simulink model "OFDMmodel_synch_18B1"  (R2025b)
settings: Solver=VariableStepAuto  StartTime=0.0  StopTime=inf  RelTol=1e-3
values from neighbouring files (symbols this model uses):
  BandasG = NFFT/4-4    (= 12)    [InitOFDM.m]
  Carriers = 1:NFFT    [InitOFDM.m]
  ChannEstData = PHI(DataCarrierIn,:)*Ainv    [InitOFDM.m]
  CP = 16    [InitOFDM.m]    (also in OFDMwideband_BEM2D.m = 32)
  DataCarrierIn = Carriers    [InitOFDM.m]
  DataCarriers = numel(DataCarrierIn)    [InitOFDM.m]
  DataCarriersFrame = DataCarriers*FrameSize    [InitOFDM.m]
  FrameSize = 40    [InitOFDM.m]
  FrameTime = Tsymbol*(FrameSize+2)    (= 0.000168)    [InitOFDM.m]
  NFFT = 64    [InitOFDM.m]    (also in OFDMwideband_BEM2D.m = 256)
  PilotIndex = UsedIndex(2:floor(numel(UsedIndex)/10):end)    [InitOFDM.m]
  pilots = randsrc(numel(PilotIndex),1,[-1 1 1i 1i])*.71    [InitOFDM.m]
  PreambuloFrec = zeros(64,1)    [InitOFDM.m]    (also in Preambulo.mat = [0 0 0 0 0 0 0 0 4 0 0 0 ... (64 elements, 64x1)])
  Ts = 1/Fs    (= 5e-08)    [InitOFDM.m]    (also in OFDMwideband_BEM2D.m = 1e-07)
undefined symbols (not defined in the file or in its folder): get, ifftshift, jet, LogicIndex, Low, magnitude
libraries: simulink x5, dspsigops x5, dspxfrm3 x4, commrflib2 x2, commchan3 x1, dspobslib x1, commrandsrc3 x1, commdigbbndam3 x1, dspswit3 x1, dspmathops x1
settings Model: Creator=Fernando  LastModifiedBy=gonzalogutierrez
settings SolverCC: AlgebraicLoopSolver=TrustRegion
settings DataIOCC: LimitDataPoints=on  MaxDataPoints=1  DSMLogging=off  SaveTime=off
settings DebuggingCC: UnconnectedInputMsg=warning  UnconnectedOutputMsg=warning  UnconnectedLineMsg=warning  ArithmeticOperatorsInVariantConditions=warning
settings ModelReferenceCC: EnableRefExpFcnMdlSchedulingChecks=on
settings SFSimCC: CustomCodeUndefinedFunction=UseInterfaceOnly
settings RTWCC: GPUComputeCapability=3.5

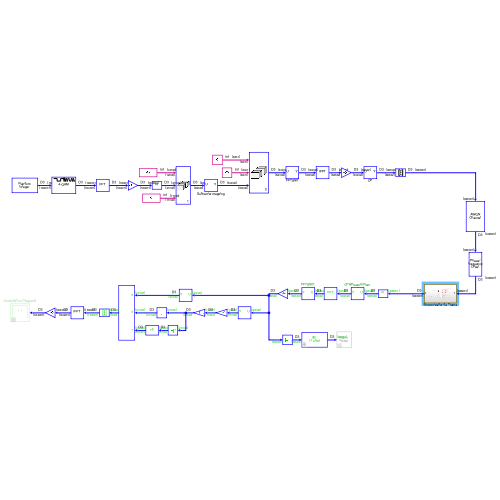
[thumbnail: Simulink's stored preview of the top-level diagram]
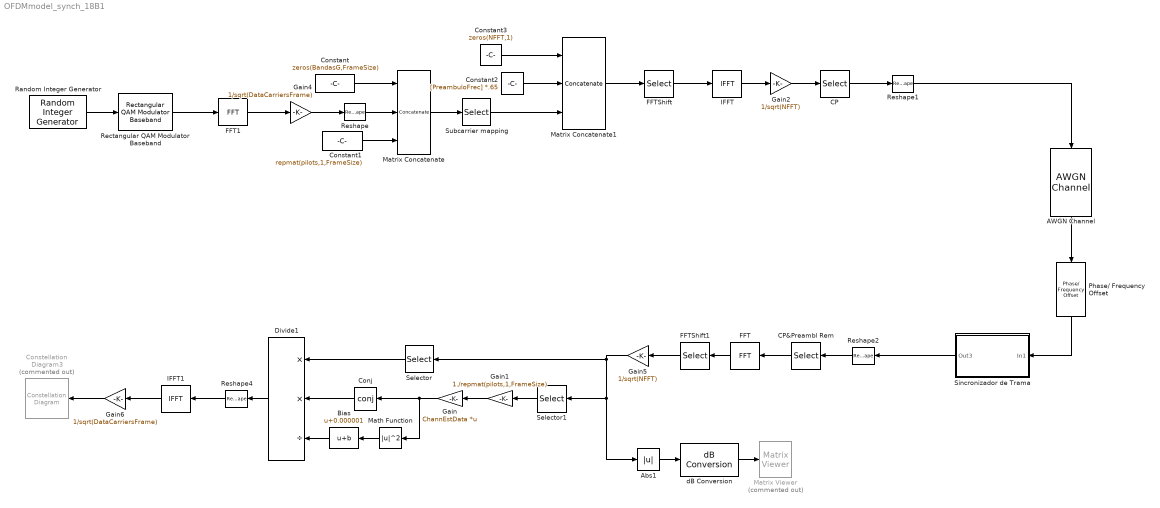
== system OFDMmodel_synch_18B1 ==
  AWGN Channel : commchan3/AWGN Channel  LegacyMode=on  NoiseMethod="Signal to noise ratio  (SNR)"  noiseMode="Signal to noise ratio  (SNR)"  EbNo=10  EsNo=10  SNR=30  BitsPerSymbol=1  SignalPower=1  SpecifySymbolPeriod=off  SamplesPerSymbol=1  SymbolPeriod=1  VarianceSource=Parameter  Variance=1  RandomStream=Global stream  Seed=67  SimulateUsing=Code generation
  Abs1 : Abs  SaturateOnIntegerOverflow=off
  Bias : Bias  Bias=0.000001  SaturateOnIntegerOverflow=off
  CP : Selector  NumberOfDimensions=2  InputPortWidth=NFFT  IndexOptions=Index vector (dialog),Select all  Indices=[NFFT-CP+1:NFFT 1:NFFT],1  OutputSizes=1,1
  CP&Preambl Rem : Selector  NumberOfDimensions=2  InputPortWidth=NFFT+CP  IndexOptions=Starting index (dialog),Starting index (dialog)  Indices=CP+1,2  OutputSizes=NFFT,FrameSize
  Conj : Math  Operator=conj  SignedPower=on
  Constant : Constant  Value=zeros(BandasG,FrameSize)  VectorParams1D=off
  Constant1 : Constant  Value=repmat(pilots,1,FrameSize)  VectorParams1D=off
  Constant2 : Constant  Value=[PreambuloFrec] *.65  VectorParams1D=off
  Constant3 : Constant  Value=zeros(NFFT,1)  VectorParams1D=off
  Constellation Diagram3 : ConstellationDiagram  Commented=on  DefaultConfigurationName=comm.scopes.ConstellationDiagramBlockCfg
  Divide1 : Product  Inputs=**/
  FFT : dspxfrm3/FFT  FFTImplementation=Auto  CompMethod=Table lookup  TableOpt=NEW  TableOptActive=Speed  BitRevOrder=off  Normalize=off  InheritFFTLength=on  FFTLength=64  WrapInput=on  roundingMode=Floor  overflowMode=off  firstCoeffDataTypeStr=Inherit: Same word length as input  firstCoeffLastDataTypeStr=Inherit: Same word length as input  outputMin=[]  outputMax=[]
  FFT1 : dspxfrm3/FFT  FFTImplementation=Auto  CompMethod=Table lookup  TableOpt=NEW  TableOptActive=Speed  BitRevOrder=off  Normalize=off  InheritFFTLength=on  FFTLength=64  WrapInput=on  roundingMode=Floor  overflowMode=off  firstCoeffDataTypeStr=Inherit: Same word length as input  firstCoeffLastDataTypeStr=Inherit: Same word length as input  outputMin=[]  outputMax=[]
  FFTShift : Selector  NumberOfDimensions=2  InputPortWidth=NFFT  IndexOptions=Index vector (dialog),Select all  Indices=ifftshift(Carriers),1  OutputSizes=1,1
  FFTShift1 : Selector  NumberOfDimensions=2  InputPortWidth=NFFT  IndexOptions=Index vector (dialog),Select all  Indices=ifftshift(Carriers),1  OutputSizes=1,1
  Gain : Gain  Gain=ChannEstData  Multiplication=Matrix(K*u)
  Gain1 : Gain  Gain=1./repmat(pilots,1,FrameSize)
  Gain2 : Gain  Gain=1/sqrt(NFFT)
  Gain4 : Gain  Gain=1/sqrt(DataCarriersFrame)
  Gain5 : Gain  Gain=1/sqrt(NFFT)
  Gain6 : Gain  Gain=1/sqrt(DataCarriersFrame)
  IFFT : dspxfrm3/IFFT  FFTImplementation=Auto  CompMethod=Table lookup  TableOpt=NEW  TableOptActive=Speed  BitRevOrder=off  cs_in=off  Normalize=off  InheritFFTLength=on  FFTLength=64  WrapInput=on  mode=Complex  outSamplingMode=Sample based  roundingMode=Floor  overflowMode=off  firstCoeffDataTypeStr=Inherit: Same word length as input  firstCoeffLastDataTypeStr=Inherit: Same word length as input  outputMin=[]  outputMax=[]
  IFFT1 : dspxfrm3/IFFT  FFTImplementation=Auto  CompMethod=Table lookup  TableOpt=NEW  TableOptActive=Speed  BitRevOrder=off  cs_in=off  Normalize=off  InheritFFTLength=on  FFTLength=64  WrapInput=on  mode=Complex  outSamplingMode=Sample based  roundingMode=Floor  overflowMode=off  firstCoeffDataTypeStr=Inherit: Same word length as input  firstCoeffLastDataTypeStr=Inherit: Same word length as input  outputMin=[]  outputMax=[]
  Math Function : Math  Operator=magnitude^2  SignedPower=on
  Matrix Concatenate : Concatenate  NumInputs=3  Mode=Multidimensional array
  Matrix Concatenate1 : Concatenate  NumInputs=3  Mode=Multidimensional array  ConcatenateDimension=2
  Matrix Viewer : dspobslib/Matrix Viewer  Commented=on  ImageParams=off  CMapStr=jet(256)  AxisColorbar=on  AxisParams=off  AxisOrigin=Upper left corner  AxisTickMode=Auto  XTickRange=[0 1]  YTickRange=[0 1]  XLabel=X-axis  YLabel=Y-axis  ZLabel=Z-axis  FigPos=get(0,'defaultfigureposition')  AxisZoom=off
      settings: YMin=-30  YMax=-20
  Phase/ Frequency Offset : commrflib2/Phase// Frequency Offset  phaseOffset=0  freqPort=off  freqOffset=5e3
  Random Integer Generator : commrandsrc3/Random Integer Generator  SetSize=ConstSize  SeedSource=Auto  Seed=0  SampleTime=FrameTime/(DataCarriers*FrameSize)  SamplesPerFrame=DataCarriers*FrameSize  OutputDataType=double  SimulateUsing=Interpreted execution
  Rectangular QAM Modulator Baseband : commdigbbndam3/Rectangular QAM Modulator Baseband  M=ConstSize  InType=Integer  Enc=Gray  Mapping=[0:15]  PowType=Average Power  MinDist=2  AvgPow=1  PeakPow=1  Ph=0  outDtype=double  outWordLen=16  outUDDataType=sfix(16)  outFracLenMode=Best precision  outFracLen=15  outDataTypeStr=double  outLastDataTypeStr=double
  Reshape : Reshape  OutputDimensionality=Customize  OutputDimensions=[DataCarriers,FrameSize]
  Reshape1 : Reshape  OutputDimensionality=Column vector (2-D)  OutputDimensions=[DataCarriers,FrameSize]
  Reshape2 : Reshape  OutputDimensionality=Customize  OutputDimensions=[NFFT+CP,FrameSize+2]
  Reshape4 : Reshape  OutputDimensionality=Column vector (2-D)  OutputDimensions=[DataCarriers,FrameSize]
  Selector : Selector  NumberOfDimensions=2  InputPortWidth=NFFT  IndexOptions=Index vector (dialog),Select all  Indices=DataCarrierIn,1  OutputSizes=1,1
  Selector1 : Selector  NumberOfDimensions=2  InputPortWidth=NFFT  IndexOptions=Index vector (dialog),Select all  Indices=PilotIndex,1  OutputSizes=1,1
  Sincronizador de Trama : Subsystem
  Subcarrier mapping : Selector  NumberOfDimensions=2  InputPortWidth=NFFT  IndexOptions=Index vector (dialog),Select all  Indices=LogicIndex,1  OutputSizes=1,1
  dB Conversion : dspmathops/dB Conversion  dBtype=dB  intype=Amplitude  R=1  fuzz=off
  wires:
  Constant/1 -> Matrix Concatenate/1
  Matrix Concatenate/1 -> Subcarrier mapping/1
  IFFT/1 -> Gain2/1
  CP/1 -> Reshape1/1
  Constant1/1 -> Matrix Concatenate/3
  Selector1/1 -> Gain1/1
  Selector/1 -> Divide1/1
  Random Integer Generator/1 -> Rectangular QAM Modulator Baseband/1
  Gain2/1 -> CP/1
  FFT/1 -> FFTShift1/1
  FFTShift1/1 -> Gain5/1
  Conj/1 -> Divide1/2
  Gain/1 -> Math Function/1, Conj/1
  Bias/1 -> Divide1/3
  Math Function/1 -> Bias/1
  Divide1/1 -> Reshape4/1
  CP&Preambl Rem/1 -> FFT/1
  Reshape/1 -> Matrix Concatenate/2
  Abs1/1 -> dB Conversion/1
  Matrix Concatenate1/1 -> FFTShift/1
  FFTShift/1 -> IFFT/1
  Constant2/1 -> Matrix Concatenate1/2
  Constant3/1 -> Matrix Concatenate1/1
  dB Conversion/1 -> Matrix Viewer/1
  Gain5/1 -> Selector1/1, Abs1/1, Selector/1
  Gain1/1 -> Gain/1
  Rectangular QAM Modulator Baseband/1 -> FFT1/1
  FFT1/1 -> Gain4/1
  IFFT1/1 -> Gain6/1
  Gain4/1 -> Reshape/1
  Gain6/1 -> Constellation Diagram3/1
  Reshape4/1 -> IFFT1/1
  Reshape2/1 -> CP&Preambl Rem/1
  Subcarrier mapping/1 -> Matrix Concatenate1/3
  Reshape1/1 -> AWGN Channel/1
  AWGN Channel/1 -> Phase/ Frequency Offset/1
  Phase/ Frequency Offset/1 -> Sincronizador de Trama/1(In1)
  Sincronizador de Trama/1(Out3) -> Reshape2/1

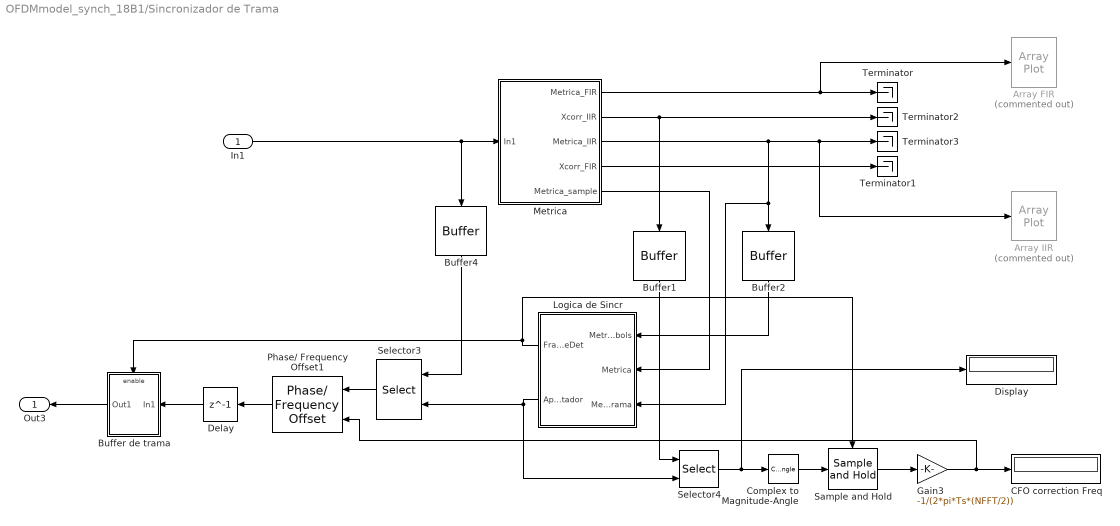
== system OFDMmodel_synch_18B1/Sincronizador de Trama ==
  In1 : Inport
  Array FIR : ArrayPlot  Commented=on  WindowPosition=[481 42 958 954]  AxesScaling=Manual  YLimits=[-0.125,1.125]  ShowGrid=off  ChannelNames="[\"\"]"  DefaultConfigurationName=dsp.scopes.ArrayPlotBlockSpecification
  Array IIR : ArrayPlot  Commented=on  WindowPosition=[241.000000,-27.000000,958.000000,954.000000,]  ScopeFrameLocation=window  AxesScaling=Manual  YLimits=[-0.125,1.125]  ShowGrid=off  ChannelNames="[\"\"]"  DefaultConfigurationName=dsp.scopes.ArrayPlotBlockSpecification
  Buffer de trama : Subsystem
  Buffer1 : Buffer  N=2*(NFFT+CP)  V=NFFT+CP  OutputFrames=off
  Buffer2 : Buffer  N=2*(NFFT+CP)  V=NFFT+CP  OutputFrames=off
  Buffer4 : Buffer  N=3*(NFFT+CP)  V=2*(NFFT+CP)  OutputFrames=off
  CFO correction Freq : Display
  Complex to Magnitude-Angle : ComplexToMagnitudeAngle  Output=Angle
  Delay : Delay  DelayLength=1
  Display : Display
  Gain3 : Gain  Gain=-1/(2*pi*Ts*(NFFT/2))
  Logica de Sincr : Subsystem
  Metrica : Subsystem
  Phase/ Frequency Offset1 : commrflib2/Phase// Frequency Offset  phaseOffset=0  freqPort=on  freqOffset=16e3
  Sample and Hold : dspsigops/Sample and Hold  trig=Rising edge  initCond=0  latchinput=off
  Selector3 : Selector  InputPortWidth=3*(NFFT+CP)  IndexOptions=Starting index (port)  Indices=[1 3]  OutputSizes=NFFT+CP
  Selector4 : Selector  InputPortWidth=2*(NFFT+CP)  IndexOptions=Index vector (port)  Indices=[1 3]  OutputSizes=1
  Terminator{,1..3} (4 alike) : Terminator
  Out3 : Outport
  wires:
  Phase/ Frequency Offset1/1 -> Delay/1
  Gain3/1 -> Phase/ Frequency Offset1/2, CFO correction Freq/1
  Buffer1/1 -> Selector4/1
  Logica de Sincr/2(Apuntador) -> Selector4/2, Selector3/2
  Sample and Hold/1 -> Gain3/1
  Logica de Sincr/1(FrameDet) -> Buffer de trama/Enable, Sample and Hold/Trigger
  Buffer4/1 -> Selector3/1
  Buffer2/1 -> Logica de Sincr/1(Metrica_2Symbols)
  Complex to Magnitude-Angle/1 -> Sample and Hold/1
  Selector3/1 -> Phase/ Frequency Offset1/1
  Metrica/2(Xcorr_IIR) -> Buffer1/1, Terminator2/1
  Delay/1 -> Buffer de trama/1(In1)
  Selector4/1 -> Display/1, Complex to Magnitude-Angle/1
  In1/1 -> Metrica/1(In1), Buffer4/1
  Metrica/3(Metrica_IIR) -> Logica de Sincr/3(Metrica_trama), Buffer2/1, Array IIR/1, Terminator3/1
  Buffer de trama/1(Out1) -> Out3/1
  Metrica/4(Xcorr_FIR) -> Terminator1/1
  Metrica/1(Metrica_FIR) -> Terminator/1, Array FIR/1
  Metrica/5(Metrica_sample) -> Logica de Sincr/2(Metrica)

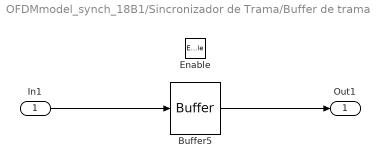
== system OFDMmodel_synch_18B1/Sincronizador de Trama/Buffer de trama ==
  In1 : Inport
  Enable : EnablePort  ZeroCross=off
  Buffer5 : Buffer  N=(NFFT+CP)*(FrameSize+2)  OutputFrames=off
  Out1 : Outport
  wires:
  In1/1 -> Buffer5/1
  Buffer5/1 -> Out1/1

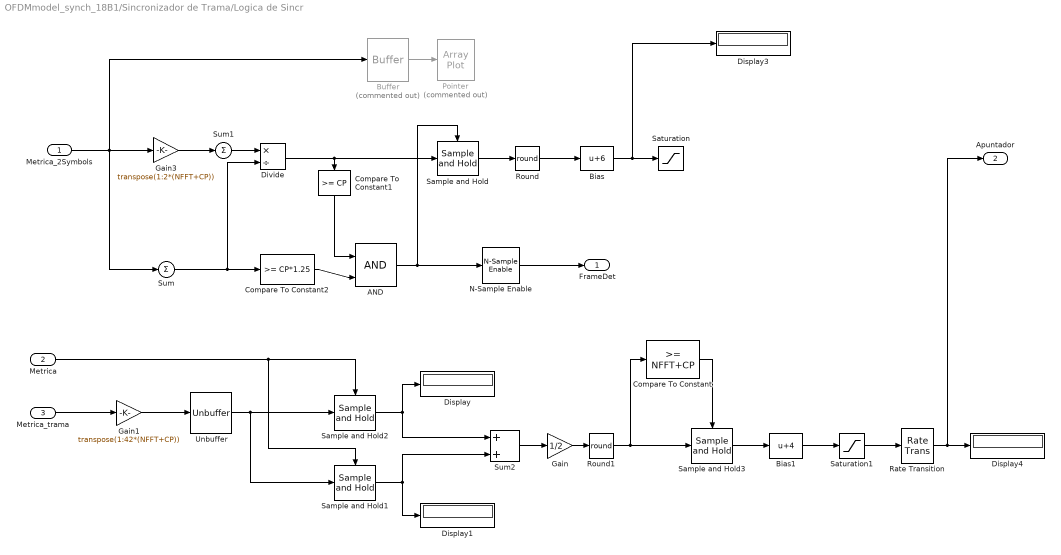
== system OFDMmodel_synch_18B1/Sincronizador de Trama/Logica de Sincr ==
  Metrica_2Symbols : Inport
  Metrica : Inport  Port=2
  Metrica_trama : Inport  Port=3
  AND : Logic  IconShape=distinctive  AllPortsSameDT=off  OutDataTypeStr=boolean
  Bias : Bias  Bias=6  SaturateOnIntegerOverflow=off
  Bias1 : Bias  Bias=4  SaturateOnIntegerOverflow=off
  Buffer : Buffer  Commented=on  N=2*(NFFT + CP)  OutputFrames=off
  Compare To Constant : simulink/Logic and Bit Operations/Compare To Constant  relop=>=  const=NFFT+CP  OutDataTypeStr=boolean
  Compare To Constant1 : simulink/Logic and Bit Operations/Compare To Constant  relop=>=  const=CP  OutDataTypeStr=boolean  ZeroCross=off
  Compare To Constant2 : simulink/Logic and Bit Operations/Compare To Constant  relop=>=  const=CP*1.25  OutDataTypeStr=boolean  ZeroCross=off
  Display{,1,3..4} (4 alike) : Display
  Divide : Product  Inputs=*/
  Gain : Gain  Gain=1/2
  Gain1 : Gain  Gain=transpose(1:42*(NFFT+CP))
  Gain3 : Gain  Gain=transpose(1:2*(NFFT+CP))
  N-Sample Enable : dspswit3/N-Sample Enable  N=FrameSize+1  ActiveLevel=Low (0)  reset=on  TriggerType=Rising edge  Ts=1  DataType=Logical
  Pointer : ArrayPlot  Commented=on  WindowPosition=[481 42 958 954]  AxesScaling=Manual  YLimits=[-16.5,168.5]  ShowGrid=off  ChannelNames="[\"\"]"  DefaultConfigurationName=dsp.scopes.ArrayPlotBlockSpecification
  Rate Transition : RateTransition  OutPortSampleTime=4e-6
  Round : Rounding  Operator=round
  Round1 : Rounding  Operator=round
  Sample and Hold : dspsigops/Sample and Hold  trig=Rising edge  initCond=0  latchinput=off
  Sample and Hold1 : dspsigops/Sample and Hold  trig=Falling edge  initCond=0  latchinput=off
  Sample and Hold2 : dspsigops/Sample and Hold  trig=Rising edge  initCond=0  latchinput=off
  Sample and Hold3 : dspsigops/Sample and Hold  trig=Rising edge  initCond=0  latchinput=off
  Saturation : Saturate  UpperLimit=2*(NFFT+CP)+1  LowerLimit=1
  Saturation1 : Saturate  UpperLimit=2*(NFFT+CP)+1  LowerLimit=1
  Sum : Sum  Inputs=+
  Sum1 : Sum  Inputs=+
  Sum2 : Sum
  Unbuffer : Unbuffer
  FrameDet : Outport
  Apuntador : Outport  Port=2
  wires:
  Metrica_2Symbols/1 -> Sum/1, Buffer/1, Gain3/1
  Sum/1 -> Divide/2, Compare To Constant2/1
  Gain3/1 -> Sum1/1
  AND/1 -> Sample and Hold/Trigger, N-Sample Enable/1
  Round/1 -> Bias/1
  Sample and Hold/1 -> Round/1
  Sum1/1 -> Divide/1
  N-Sample Enable/1 -> FrameDet/1
  Bias/1 -> Display3/1, Saturation/1
  Compare To Constant2/1 -> AND/2
  Compare To Constant1/1 -> AND/1
  Buffer/1 -> Pointer/1
  Divide/1 -> Sample and Hold/1, Compare To Constant1/1
  Metrica_trama/1 -> Gain1/1
  Sample and Hold1/1 -> Sum2/2, Display1/1
  Sample and Hold2/1 -> Sum2/1, Display/1
  Metrica/1 -> Sample and Hold2/Trigger, Sample and Hold1/Trigger
  Sum2/1 -> Gain/1
  Gain1/1 -> Unbuffer/1
  Unbuffer/1 -> Sample and Hold1/1, Sample and Hold2/1
  Gain/1 -> Round1/1
  Sample and Hold3/1 -> Bias1/1
  Compare To Constant/1 -> Sample and Hold3/Trigger
  Round1/1 -> Compare To Constant/1, Sample and Hold3/1
  Bias1/1 -> Saturation1/1
  Saturation1/1 -> Rate Transition/1
  Rate Transition/1 -> Apuntador/1, Display4/1

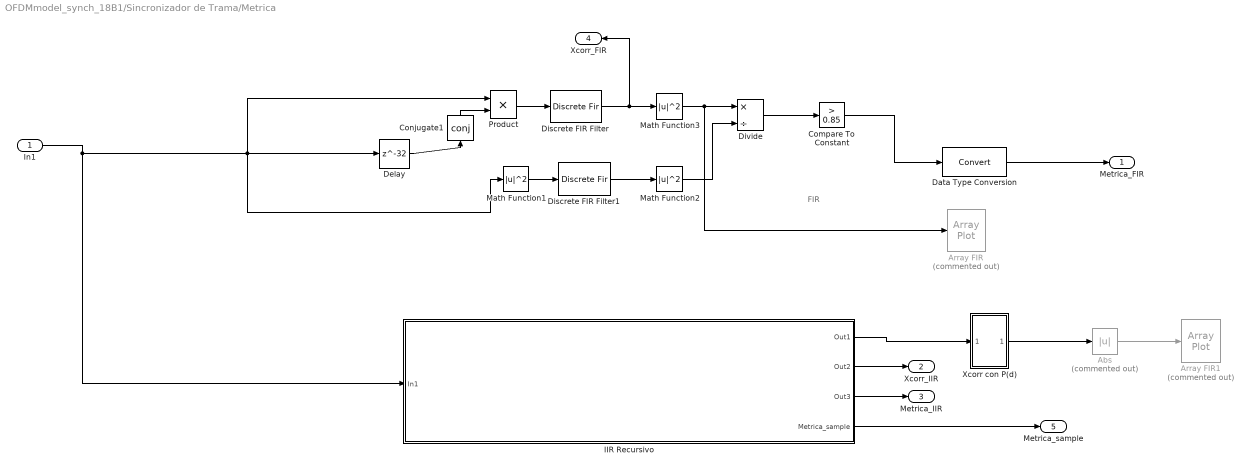
== system OFDMmodel_synch_18B1/Sincronizador de Trama/Metrica ==
  note: FIR
  In1 : Inport
  Abs : Abs  Commented=on  SaturateOnIntegerOverflow=off
  Array FIR : ArrayPlot  Commented=on  WindowPosition=[480 -51 958 954]  AxesScaling=Manual  YLimits=[-821.624,7394.62]  ShowGrid=off  ChannelNames="[\"\"]"  DefaultConfigurationName=dsp.scopes.ArrayPlotBlockSpecification
  Array FIR1 : ArrayPlot  Commented=on  WindowPosition=[2 -5 1920 963]  AxesScaling=Manual  YLimits=[-16377.7,109222]  ShowGrid=off  ChannelNames="[\"\"]"  DefaultConfigurationName=dsp.scopes.ArrayPlotBlockSpecification
  Compare To Constant : simulink/Logic and Bit Operations/Compare To Constant  relop=>  const=0.85  OutDataTypeStr=uint8  ZeroCross=off
  Conjugate1 : Math  Operator=conj  SignedPower=on  RndMeth=Zero
  Data Type Conversion : DataTypeConversion  SaturateOnIntegerOverflow=off  RndMeth=Floor
  Delay : Delay  DelayLength=32  InputProcessing=Columns as channels (frame based)
  Discrete FIR Filter : DiscreteFir  Coefficients=ones(1,32)  InputProcessing=Columns as channels (frame based)
  Discrete FIR Filter1 : DiscreteFir  Coefficients=0.5*ones(1,NFFT)  InputProcessing=Columns as channels (frame based)
  Divide : Product  Inputs=*/
  IIR Recursivo : Subsystem
  Math Function1 : Math  Operator=magnitude^2  SignedPower=on
  Math Function2 : Math  Operator=magnitude^2  SignedPower=on
  Math Function3 : Math  Operator=magnitude^2  SignedPower=on
  Product : Product
  Xcorr con P(d) : Subsystem
  Metrica_FIR : Outport
  Xcorr_IIR : Outport  Port=2
  Metrica_IIR : Outport  Port=3
  Xcorr_FIR : Outport  Port=4
  Metrica_sample : Outport  Port=5
  wires:
  Delay/1 -> Conjugate1/1
  Discrete FIR Filter/1 -> Xcorr_FIR/1, Math Function3/1
  Product/1 -> Discrete FIR Filter/1
  Math Function1/1 -> Discrete FIR Filter1/1
  Compare To Constant/1 -> Data Type Conversion/1
  Discrete FIR Filter1/1 -> Math Function2/1
  Math Function3/1 -> Array FIR/1, Divide/1
  Math Function2/1 -> Divide/2
  Data Type Conversion/1 -> Metrica_FIR/1
  Conjugate1/1 -> Product/2
  Divide/1 -> Compare To Constant/1
  In1/1 -> IIR Recursivo/1(In1), Product/1, Delay/1, Math Function1/1
  IIR Recursivo/1(Out1) -> Xcorr con P(d)/1(In1)
  IIR Recursivo/2(Out2) -> Xcorr_IIR/1
  IIR Recursivo/3(Out3) -> Metrica_IIR/1
  Xcorr con P(d)/1(Out1) -> Abs/1
  Abs/1 -> Array FIR1/1
  IIR Recursivo/4(Metrica_sample) -> Metrica_sample/1

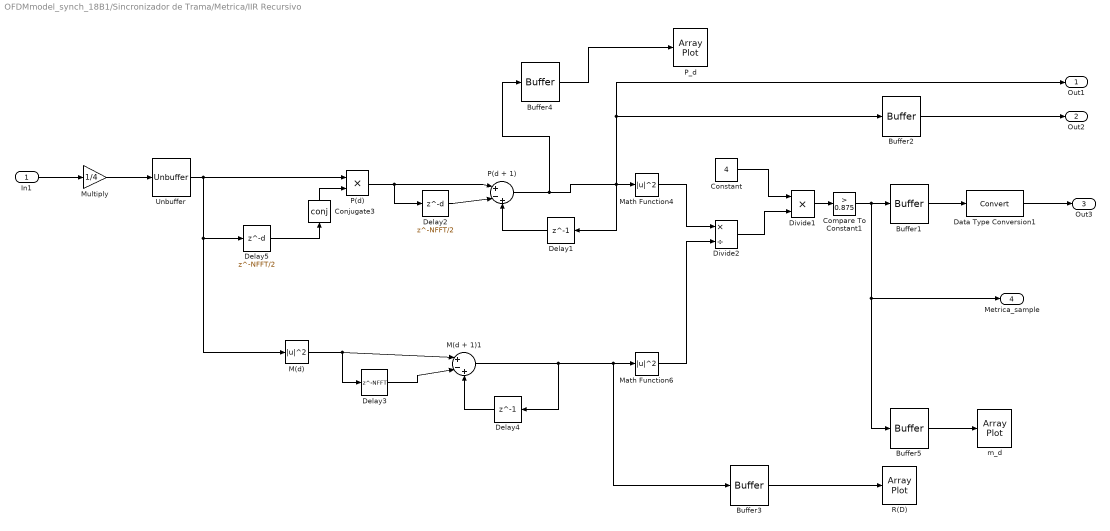
== system OFDMmodel_synch_18B1/Sincronizador de Trama/Metrica/IIR Recursivo ==
  In1 : Inport
  Buffer{1..5} (5 alike) : Buffer  N=(NFFT + CP) * 42  OutputFrames=off
  Compare To Constant1 : simulink/Logic and Bit Operations/Compare To Constant  relop=>  const=0.875  OutDataTypeStr=uint8  ZeroCross=off
  Conjugate3 : Math  Operator=conj  SignedPower=on  RndMeth=Zero
  Constant : Constant  Value=4
  Data Type Conversion1 : DataTypeConversion  SaturateOnIntegerOverflow=off  RndMeth=Floor
  Delay1 : Delay  DelayLength=1
  Delay2 : Delay  DelayLength=NFFT/2  InputProcessing=Columns as channels (frame based)
  Delay3 : Delay  DelayLength=NFFT
  Delay4 : Delay  DelayLength=1
  Delay5 : Delay  DelayLength=NFFT/2  InputProcessing=Columns as channels (frame based)
  Divide1 : Product  Inputs=**
  Divide2 : Product  Inputs=*/
  M(d + 1)1 : Sum  Inputs=|+-+
  M(d) : Math  Operator=magnitude^2  SignedPower=on
  Math Function4 : Math  Operator=magnitude^2  SignedPower=on
  Math Function6 : Math  Operator=magnitude^2  SignedPower=on
  Multiply : Gain  Gain=1/4
  P(d + 1) : Sum  Inputs=|+-+
  P(d) : Product
  P_d : ArrayPlot  WindowPosition=[0.000000,1.000000,1440.000000,842.000000,]  Visible=on  ScopeFrameLocation=window  AxesScaling=Manual  MaximizeAxes=Off  YLimits=[-0.9249 5.7278]  ShowGrid=off  ChannelNames="[\"\"]"  DefaultConfigurationName=dsp.scopes.ArrayPlotBlockSpecification
  R(D) : ArrayPlot  WindowPosition=[721.000000,1.000000,720.000000,842.000000,]  Visible=on  ScopeFrameLocation=window  AxesScaling=Manual  YLimits=[7.313850160256411 10.478150160256412]  ShowGrid=off  ChannelNames="[\"\"]"  DefaultConfigurationName=dsp.scopes.ArrayPlotBlockSpecification
  Unbuffer : Unbuffer
  m_d : ArrayPlot  WindowPosition=[1.000000,1.000000,1440.000000,842.000000,]  Visible=on  ScopeFrameLocation=window  AxesScaling=Manual  YLimits=[-0.116212,1.04604]  ShowGrid=off  ChannelNames="[\"\"]"  DefaultConfigurationName=dsp.scopes.ArrayPlotBlockSpecification
  Out1 : Outport
  Out2 : Outport  Port=2
  Out3 : Outport  Port=3
  Metrica_sample : Outport  Port=4
  wires:
  P(d + 1)/1 -> Buffer4/1, Out1/1, Buffer2/1, Math Function4/1, Delay1/1
  M(d)/1 -> Delay3/1, M(d + 1)1/1
  Unbuffer/1 -> P(d)/1, M(d)/1, Delay5/1
  Delay4/1 -> M(d + 1)1/3
  Buffer1/1 -> Data Type Conversion1/1
  Math Function6/1 -> Divide2/2
  P(d)/1 -> Delay2/1, P(d + 1)/1
  Compare To Constant1/1 -> Buffer5/1, Metrica_sample/1, Buffer1/1
  Divide2/1 -> Divide1/2
  Divide1/1 -> Compare To Constant1/1
  Buffer2/1 -> Out2/1
  Buffer3/1 -> R(D)/1
  Delay1/1 -> P(d + 1)/3
  Delay3/1 -> M(d + 1)1/2
  Delay5/1 -> Conjugate3/1
  Math Function4/1 -> Divide2/1
  Conjugate3/1 -> P(d)/2
  Delay2/1 -> P(d + 1)/2
  Constant/1 -> Divide1/1
  In1/1 -> Multiply/1
  Data Type Conversion1/1 -> Out3/1
  M(d + 1)1/1 -> Buffer3/1, Math Function6/1, Delay4/1
  Buffer4/1 -> P_d/1
  Buffer5/1 -> m_d/1
  Multiply/1 -> Unbuffer/1

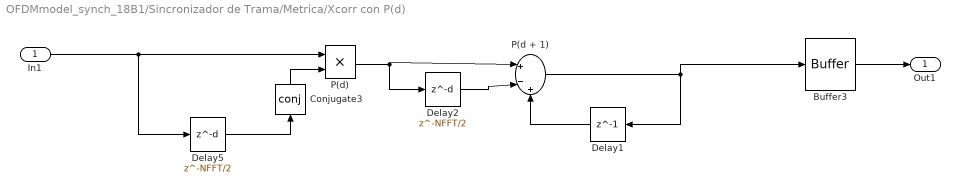
== system OFDMmodel_synch_18B1/Sincronizador de Trama/Metrica/Xcorr con P(d) ==
  In1 : Inport
  Buffer3 : Buffer  N=(NFFT + CP) * 42  OutputFrames=off
  Conjugate3 : Math  Operator=conj  SignedPower=on  RndMeth=Zero
  Delay1 : Delay  DelayLength=1
  Delay2 : Delay  DelayLength=NFFT/2  InputProcessing=Columns as channels (frame based)
  Delay5 : Delay  DelayLength=NFFT/2  InputProcessing=Columns as channels (frame based)
  P(d + 1) : Sum  Inputs=|+-+
  P(d) : Product
  Out1 : Outport
  wires:
  Conjugate3/1 -> P(d)/2
  P(d)/1 -> Delay2/1, P(d + 1)/1
  Delay2/1 -> P(d + 1)/2
  Delay5/1 -> Conjugate3/1
  Delay1/1 -> P(d + 1)/3
  In1/1 -> P(d)/1, Delay5/1
  Buffer3/1 -> Out1/1
  P(d + 1)/1 -> Delay1/1, Buffer3/1
